simulink model "B3_AHB"  (R2022b)
settings: Solver=FixedStepDiscrete  StartTime=0.0  StopTime=60  FixedStep=Ts  RelTol=1e-3
values from neighbouring files (symbols this model uses):
  LUX_AHB = 50    [build_B3_AHB.m]
  T_REARM = 2    [build_B3_AHB.m]
  Ts = 0.01    [build_B2_AutoHeadlamp.m]    (also in build_B3_AHB.m)
  V_AHB_OFF = 30    [build_B3_AHB.m]
  V_AHB_ON = 40    [build_B3_AHB.m]
settings Model: Creator=LENOVO  LastModifiedBy=LENOVO

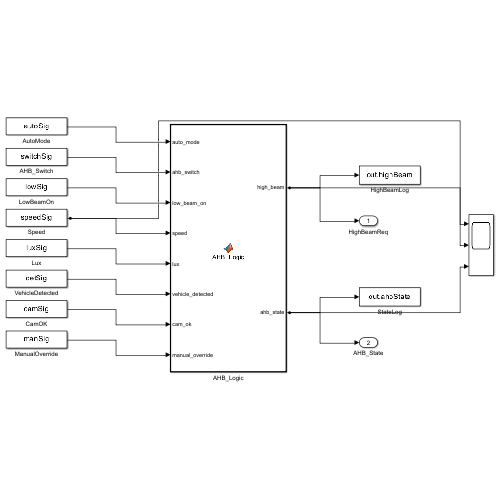
[thumbnail: Simulink's stored preview of the top-level diagram]
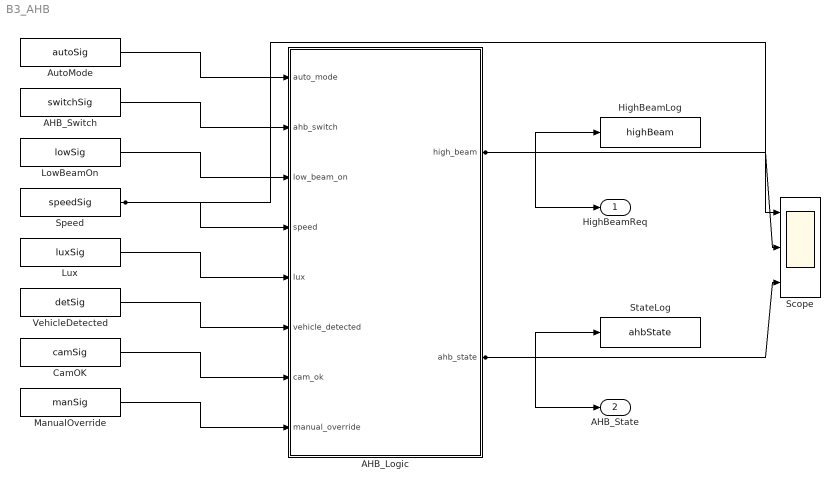
== system B3_AHB ==
  AHB_Logic : MATLAB Function  TreatAsAtomicUnit=on
  AHB_Switch : FromWorkspace  VariableName=switchSig  SampleTime=Ts  Interpolate=off  OutputAfterFinalValue=Holding final value
  AutoMode : FromWorkspace  VariableName=autoSig  SampleTime=Ts  Interpolate=off  OutputAfterFinalValue=Holding final value
  CamOK : FromWorkspace  VariableName=camSig  SampleTime=Ts  Interpolate=off  OutputAfterFinalValue=Holding final value
  HighBeamLog : ToWorkspace  VariableName=highBeam  SaveFormat=Timeseries  SampleTime=-1
  LowBeamOn : FromWorkspace  VariableName=lowSig  SampleTime=Ts  Interpolate=off  OutputAfterFinalValue=Holding final value
  Lux : FromWorkspace  VariableName=luxSig  SampleTime=Ts  OutputAfterFinalValue=Holding final value
  ManualOverride : FromWorkspace  VariableName=manSig  SampleTime=Ts  Interpolate=off  OutputAfterFinalValue=Holding final value
  Scope : Scope  NumInputPorts=3
  Speed : FromWorkspace  VariableName=speedSig  SampleTime=Ts  OutputAfterFinalValue=Holding final value
  StateLog : ToWorkspace  VariableName=ahbState  SaveFormat=Timeseries  SampleTime=-1
  VehicleDetected : FromWorkspace  VariableName=detSig  SampleTime=Ts  Interpolate=off  OutputAfterFinalValue=Holding final value
  HighBeamReq : Outport
  AHB_State : Outport  Port=2
  wires:
  AutoMode/1 -> AHB_Logic/1(auto_mode)
  AHB_Switch/1 -> AHB_Logic/2(ahb_switch)
  LowBeamOn/1 -> AHB_Logic/3(low_beam_on)
  Speed/1 -> AHB_Logic/4(speed), Scope/1
  Lux/1 -> AHB_Logic/5(lux)
  VehicleDetected/1 -> AHB_Logic/6(vehicle_detected)
  CamOK/1 -> AHB_Logic/7(cam_ok)
  ManualOverride/1 -> AHB_Logic/8(manual_override)
  AHB_Logic/1(high_beam) -> HighBeamLog/1, HighBeamReq/1, Scope/2
  AHB_Logic/2(ahb_state) -> StateLog/1, AHB_State/1, Scope/3

== matlab function B3_AHB/AHB_Logic ==
  data: auto_mode input; high_beam output; ahb_switch input; low_beam_on input; speed input; lux input; vehicle_detected input; cam_ok input; manual_override input; ahb_state output; Ts parameter; V_AHB_ON parameter; V_AHB_OFF parameter; LUX_AHB parameter; T_REARM parameter
function [high_beam, ahb_state] = AHB_Logic(auto_mode, ahb_switch, low_beam_on, speed, lux, vehicle_detected, cam_ok, manual_override, Ts, V_AHB_ON, V_AHB_OFF, LUX_AHB, T_REARM)
%#codegen
% B3 - Auto High Beam (AHB) : feux de route automatiques
% ahb_state : 0 = OFF (non disponible), 1 = READY (disponible, route non libre)
%             2 = ACTIVE (feux de route), 3 = PAUSE (action manuelle), 4 = FAULT (camera)
persistent spd_ok clear_cnt hb
if isempty(spd_ok)
    spd_ok = false; clear_cnt = 0; hb = false;
end
% --- Hysteresis de vitesse (REQ-LSC-13) : ON a 40 km/h, OFF sous 30 km/h
if speed >= V_AHB_ON
    spd_ok = true;
elseif speed < V_AHB_OFF
    spd_ok = false;
end
% --- Conditions de disponibilite (REQ-LSC-10)
avail = auto_mode && ahb_switch && low_beam_on && spd_ok && (lux < LUX_AHB);

if ~cam_ok                          % camera en defaut -> etat sur (REQ-LSC-14)
    hb = false; clear_cnt = 0; st = 4;
elseif manual_override              % le conducteur est prioritaire (REQ-LSC-15)
    hb = false; clear_cnt = 0; st = 3;
elseif ~avail                       % conditions non reunies
    hb = false; clear_cnt = 0; st = 0;
elseif vehicle_detected             % usager detecte -> croisement immediat (REQ-LSC-11)
    hb = false; clear_cnt = 0; st = 1;
else                                % route libre : confirmation pendant T_REARM (REQ-LSC-12)
    clear_cnt = min(clear_cnt + Ts, 100);
    if clear_cnt > T_REARM + Ts/2
        hb = true;
    end
    if hb
        st = 2;
    else
        st = 1;
    end
end
high_beam = hb;
ahb_state = uint8(st);
